simulink model "ADCSSimulator"  (R2024a)
settings: Solver=ode4  StartTime=0.0  StopTime=600  FixedStep=0.01  MaxStep=0.1  RelTol=1e-3  AbsTol=1e-3
values from neighbouring files (symbols this model uses):
  ActuatorAllocationMatrix = ActuatorPhysicalMatrix' * inv(ActuatorPhysicalMatrix * ActuatorPhysicalMatrix')    [set_Init.m]
  ActuatorPhysicalMatrix = [1, 0, 0, 0 ... (first row only)    [set_Init.m]
  albedo_irradiance = 300    [set_Init.m]
  b = 0    [set_Init.m]
  Cd = 2.2    [set_Init.m]
  h_bias = [0; 0; 0]    [set_Init.m]
  J = 4.0e-3 / 628    (= 6.36942675159e-06)    [set_Init.m]
  k_Bdot = ((4 * pi * 0.5236 * 0.0055) / (5677.2 * (4.5e-5)^2))    (= 3147.8423197)    [set_Init.m]
  K_E = K_T    (= 0.0022)    [set_Init.m]
  K_T = 0.0022    [set_Init.m]
  P0 = blkdiag(P0_att, P0_bias)    [set_Init.m]
  P0_att = eye(3) * initial_variance_rad2    [set_Init.m]
  PowerVoltageBus_01 = 3.3    [set_Init.m]
  PowerVoltageBus_02 = 3.3    [set_Init.m]
  PowerVoltageBus_03 = 3.3    [set_Init.m]
  PowerVoltageBus_04 = 3.3    [set_Init.m]
  PowerVoltageBus_05 = 3.3    [set_Init.m]
  PowerVoltageBus_06 = 3.3    [set_Init.m]
  PowerVoltageBus_07 = 3.3    [set_Init.m]
  PowerVoltageBus_08 = 3.3    [set_Init.m]
  PowerVoltageBus_09 = 3.3    [set_Init.m]
  PowerVoltageBus_10 = 3.3    [set_Init.m]
  PowerVoltageBus_11 = 3.3    [set_Init.m]
  PowerVoltageBus_12 = 0.0    (= 0)    [set_Init.m]
  PowerVoltageBus_13 = 0.0    (= 0)    [set_Init.m]
  PowerVoltageBus_14 = 0.0    (= 0)    [set_Init.m]
  PowerVoltageBus_15 = 0.0    (= 0)    [set_Init.m]
  R = 2.0    (= 2)    [set_Init.m]
  ressidual_m = [3e-4; -2e-4; 1e-4]    [set_Init.m]
  solar_irradiance = 1361    [set_Init.m]
  surface_areas = [A_xy, A_yz, A_xz, A_xy, A_yz, A_xz]    [set_Init.m]
  surface_normals_body = [eye(3) -eye(3)]    [set_Init.m]
  surface_positions_body = [       hx,   0,   0 ... (first row only)    [set_Init.m]
  surface_reflectivities = [0.9 0.8 0.9 0.9 0.9 0.9]    [set_Init.m]
  Switch_01 = 1    [set_Init.m]
  Switch_02 = 1    [set_Init.m]
  Switch_03 = 1    [set_Init.m]
  Switch_04 = 1    [set_Init.m]
  Switch_05 = 1    [set_Init.m]
  Switch_06 = 1    [set_Init.m]
  Switch_07 = 1    [set_Init.m]
  Switch_08 = 1    [set_Init.m]
  Switch_09 = 1    [set_Init.m]
  Switch_10 = 1    [set_Init.m]
  Switch_11 = 1    [set_Init.m]
  Switch_12 = 0    [set_Init.m]
  Switch_13 = 0    [set_Init.m]
  Switch_14 = 0    [set_Init.m]
  Switch_15 = 0    [set_Init.m]
  visSampleTime = 0.1    [set_Init.m]
undefined symbols (not defined in the file or in its folder): attitude, Controller, epoch, IAU, juliandate, Kd, km, Kp, m, rad, s, satellite, SGP4_parameters, simulator, UKF_parameters, WMM2020
libraries: sharedtransform x27, aerolibutil x22, aerolibconvert2 x18, simulink_extras x16, matrix_library x6, aerolibtransform2 x4, vrlib x2, aerolibgravity2 x2, aerolibobsolete x1, aerolibattitudesys x1, simulink x1
(part 4 of 8)

== system ADCSSimulator/ADCS/ADCS Software/Onboard Reference Frames Transformations Manager1/Ensure Quaternion Continuity3 ==
  q_in : Inport
  Ensure Quaternion Continuity : MATLAB Function  TreatAsAtomicUnit=on
  Unit Delay : UnitDelay  InitialCondition=[1;0;0;0]  SampleTime=-1  HasFrameUpgradeWarning=on
  q_out : Outport
  wires:
  Ensure Quaternion Continuity/1(q_out) -> q_out/1, Unit Delay/1
  Unit Delay/1 -> Ensure Quaternion Continuity/2(q_prev)
  q_in/1 -> Ensure Quaternion Continuity/1(q_new)

== system ADCSSimulator/ADCS/ADCS Software/Onboard Reference Frames Transformations Manager1/Ensure Quaternion Continuity4 ==
  q_in : Inport
  Ensure Quaternion Continuity : MATLAB Function  TreatAsAtomicUnit=on
  Unit Delay : UnitDelay  InitialCondition=[1;0;0;0]  SampleTime=-1  HasFrameUpgradeWarning=on
  q_out : Outport
  wires:
  Ensure Quaternion Continuity/1(q_out) -> q_out/1, Unit Delay/1
  Unit Delay/1 -> Ensure Quaternion Continuity/2(q_prev)
  q_in/1 -> Ensure Quaternion Continuity/1(q_new)

== system ADCSSimulator/ADCS/ADCS Software/Onboard Reference Frames Transformations Manager1/Ensure Quaternion Continuity5 ==
  q_in : Inport
  Ensure Quaternion Continuity : MATLAB Function  TreatAsAtomicUnit=on
  Unit Delay : UnitDelay  InitialCondition=[1;0;0;0]  SampleTime=-1  HasFrameUpgradeWarning=on
  q_out : Outport
  wires:
  Ensure Quaternion Continuity/1(q_out) -> q_out/1, Unit Delay/1
  Unit Delay/1 -> Ensure Quaternion Continuity/2(q_prev)
  q_in/1 -> Ensure Quaternion Continuity/1(q_new)

== system ADCSSimulator/ADCS/ADCS Software/Onboard Reference Frames Transformations Manager1/ICRF to ITRF DCM Calculator ==
  note: Goal: Transformation Between ICRF (ECI) and ITRF (ECEF)
  note: **********************************************************************
      | * *
      | * I E R S B U L L E T I N - A *
      | * *
      | * Rapid Service/Prediction of Earth Orientation *
      | **********************************************************************
      | 30 September 2021 Vol. XXXIV No. 039
      | ______________________________________________________________________
      | GENERAL INFORMATION:
      | To receive this information electronically, contact:
      | ser7@maia.usno.navy.mil or use
      | <http://maia.usno.navy.mil/docrequest.html>
      | MJD = Julian Date - 2 400 000.5 days
      | UT2-UT1 = 0.022 sin(2*pi*T) - 0.012 cos(2*pi*T)
      | - 0.006 sin(4*pi*T) + 0.007 cos(4*pi*T)
      | where pi = 3.14159265... and T is the date in Besselian years.
      | TT = TAI + 32.184 seconds
      | DUT1= (UT1-UTC) transmitted with time signals
      | = -0.1 seconds beginning 17 July 2021 at 0000 UTC
      | Beginning 1 January 2017:
      | TAI-UTC = 37.000 000 seconds
  Calendar : Inport
  Bus Selector : BusSelector  OutputSignals=Modified Julian Date (day),Since Epoch (sec)
  Constant2 : Constant  Value=37
  Direction Cosine Matrix ICRF to ITRF : aerolibtransform2/Direction Cosine Matrix ECI to ECEF  red=IAU-2000/2006  year=epoch.Year  month=October  day=12  hour=epoch.Hour  min=epoch.Minute  sec=epoch.Second  deltaT=Sec  errorflag=Error  extraparamflag=on
      settings: AttributesFormatString=%<red>
  Earth Orientation Parameters : EOParameters
  ICRF to ITRF DCM : Outport
  wires:
  Earth Orientation Parameters/2 -> Direction Cosine Matrix ICRF to ITRF/3  "Polar Displacement of Earth"
  Constant2/1 -> Direction Cosine Matrix ICRF to ITRF/2
  Calendar/1 -> Bus Selector/1
  Earth Orientation Parameters/3 -> Direction Cosine Matrix ICRF to ITRF/4  "Celestial Intermediate Pole (CIP)  adjustment (radians)"
  Direction Cosine Matrix ICRF to ITRF/1 -> ICRF to ITRF DCM/1
  Bus Selector/1 -> Earth Orientation Parameters/1  "<Modified Julian Date (day)>"
  Earth Orientation Parameters/1 -> Direction Cosine Matrix ICRF to ITRF/1
  Bus Selector/2 -> Direction Cosine Matrix ICRF to ITRF/5  "<Since Epoch (sec)>"

== system ADCSSimulator/ADCS/ADCS Software/Onboard Reference Frames Transformations Manager1/Orbit to Body Transfer Matrix Calculator1 ==
  ICRF2BodyDCM : Inport
  Keplerian Elements : Inport  Port=2
  Bus Selector : BusSelector  OutputSignals=Argument of Perigee [omega] (rad),True Anomaly [nu] (rad),Inclination [i] (rad),Right Ascension [Omega] (rad)
  Interpreted MATLAB Function : MATLABFcn  MATLABFcn=[cos(u),sin(u),0; -sin(u),cos(u),0; 0,0,1]  OutputDimensions=[3,3]  Output1D=off
  Interpreted MATLAB Function1 : MATLABFcn  MATLABFcn=[1,0,0;0,cos(u),sin(u);0,-sin(u),cos(u)]  OutputDimensions=[3,3]  Output1D=off
  Interpreted MATLAB Function2 : MATLABFcn  MATLABFcn=[cos(u),sin(u),0;-sin(u),cos(u),0;0,0,1]  OutputDimensions=[3,3]  Output1D=off
  Matrix Multiply{,1..3} (4 alike) : Product  Multiplication=Matrix(*)
  RotMat : Constant  Value=[0,1,0;0,0,-1;-1,0,0]
  Sum : Sum  Inputs=|++
  Transpose : Math  Operator=transpose
  Orbit2BodyTM : Outport
  wires:
  Bus Selector/3 -> Interpreted MATLAB Function1/1  "<Inclination [i] (rad)>"
  Keplerian Elements/1 -> Bus Selector/1
  Interpreted MATLAB Function2/1 -> Matrix Multiply1/2
  Interpreted MATLAB Function/1 -> Matrix Multiply/1
  Sum/1 -> Interpreted MATLAB Function/1
  RotMat/1 -> Matrix Multiply2/1
  Matrix Multiply2/1 -> Transpose/1  "ICRF to Orbit DCM"
  ICRF2BodyDCM/1 -> Matrix Multiply3/1  "ICRF to Body DCM"
  Bus Selector/1 -> Sum/1  "<Argument of Perigee [omega] (rad)>"
  Bus Selector/2 -> Sum/2  "<True Anomaly [nu] (rad)>"
  Matrix Multiply/1 -> Matrix Multiply1/1
  Matrix Multiply3/1 -> Orbit2BodyTM/1  "Orbit to Body DCM"
  Interpreted MATLAB Function1/1 -> Matrix Multiply/2
  Bus Selector/4 -> Interpreted MATLAB Function2/1  "<Right Ascension [Omega] (rad)>"
  Matrix Multiply1/1 -> Matrix Multiply2/2  "ICRF to Orbit DCM"
  Transpose/1 -> Matrix Multiply3/2  "Orbit to ICRF DCM"

== system ADCSSimulator/ADCS/ADCS Software/Orbit Detemination/Latching Logic ==
  Satellite Postion [ICRF] (km) : Inport
  Satellite Velocity [ICRF] (km/s) : Inport  Port=2
  Clock : Clock
  MATLAB Function4 : MATLAB Function  TreatAsAtomicUnit=on
  Switch : Switch  Criteria=u2 > Threshold  SaturateOnIntegerOverflow=off  InputSameDT=off
  Unit Delay : UnitDelay  InitialCondition=zeros(6, 1)  SampleTime=-1  HasFrameUpgradeWarning=on
  x_initial : Outport
  wires:
  Satellite Velocity [ICRF] (km/s)/1 -> MATLAB Function4/2(v_eci_km_s)
  Satellite Postion [ICRF] (km)/1 -> MATLAB Function4/1(r_eci_km)
  Clock/1 -> Switch/2
  MATLAB Function4/1(x_initial) -> Switch/3
  Switch/1 -> Unit Delay/1
  Unit Delay/1 -> Switch/1, x_initial/1

== system ADCSSimulator/ADCS/ADCS Software/Orbit Detemination/Onboard Orbit Propagator  ==
  Measured Satellite Ephemeris : Inport
  Bus Creator4 : BusCreator  Inputs=4
  Bus Selector4 : BusSelector  OutputSignals=Measured Position [ITRF] (m),Measured Velocity [ITRF] (m/s)
  Orbit Propagator Numerical (Kepler-Unperturbed) : OrbitPropagator  propagator=Numerical (high precision)  startDate=juliandate(epoch.Year, epoch.Month, epoch.Day, epoch.Hour, epoch.Minute, epoch.Second)  dateOut=off  orbitType=Circular inclined  semiMajorAxis=Semi_major_axis  inclination=Inclination  raan=RAAN  argLat=Argument_of_latitude  inertialPosition=[3649700.0 3308200.0 -4676600.0]  inertialVelocity=[-2750.8 6666.4 2573.4]  fixedPosition=[-4142689.0 -2676864.7 -4669861.6]  fixedVelocity=[1452.7 -6720.7 2568.1]  customR=3396200  customMu=4.305e13  customJ2=1.0826269e-03  customOmega=4.06125949e-3
  Onboard Satellite Ephemeris [ICRF] : Outport
  wires:
  Orbit Propagator Numerical (Kepler-Unperturbed)/2 -> Bus Creator4/2  "Satellite Velocity [ICRF] (m/s)"
  Orbit Propagator Numerical (Kepler-Unperturbed)/1 -> Bus Creator4/1  "Satellite Position [ICRF] (m)"
  Bus Creator4/1 -> Onboard Satellite Ephemeris [ICRF]/1  "Onboard Satellite Ephemeris [ICRF]"
  Measured Satellite Ephemeris/1 -> Bus Selector4/1
  Bus Selector4/1 -> Bus Creator4/3  "<Measured Position [ITRF] (m)>"
  Bus Selector4/2 -> Bus Creator4/4  "<Measured Velocity [ITRF] (m/s)>"

== system ADCSSimulator/ADCS/ADCS Software/Orbit Detemination/Step Time ==
  Add : Sum  Inputs=|+-
  Clock : Clock
  Unit Delay : UnitDelay  SampleTime=-1  HasFrameUpgradeWarning=on
  dt : Outport
  wires:
  Clock/1 -> Unit Delay/1, Add/1
  Add/1 -> dt/1
  Unit Delay/1 -> Add/2

== system ADCSSimulator/ADCS/ADCS Software/Orbit Detemination/Step Time1 ==
  Add : Sum  Inputs=|+-
  Clock : Clock
  Unit Delay : UnitDelay  SampleTime=-1  HasFrameUpgradeWarning=on
  dt : Outport
  wires:
  Unit Delay/1 -> Add/2
  Add/1 -> dt/1
  Clock/1 -> Add/1, Unit Delay/1

== system ADCSSimulator/ADCS/Environment Model/Attitude Dynamics & Kynematics/sqrt ==
  u : Inport
  Dot Product : DotProduct  OutDataTypeStr=Inherit: Inherit via internal rule
  Sqrt1 : Sqrt
  sqrt(u) : Outport
  wires:
  Dot Product/1 -> Sqrt1/1
  u/1 -> Dot Product/2, Dot Product/1
  Sqrt1/1 -> sqrt(u)/1

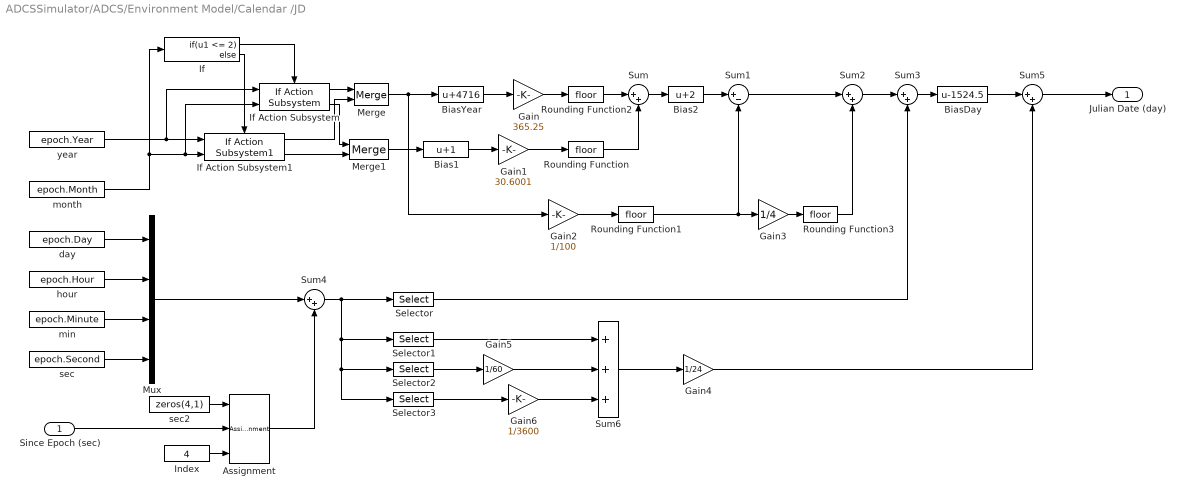
== system ADCSSimulator/ADCS/Environment Model/Calendar /JD ==
  Since Epoch (sec) : Inport  OutMin=0  PortDimensions=1
  Assignment : Assignment  IndexOptions=Index vector (port)  Indices=1  OutputSizes=1
  Bias1 : Bias  Bias=1  SaturateOnIntegerOverflow=off
  Bias2 : Bias  Bias=2  SaturateOnIntegerOverflow=off
  BiasDay : Bias  Bias=-1524.5  SaturateOnIntegerOverflow=off
  BiasYear : Bias  Bias=4716  SaturateOnIntegerOverflow=off
  Gain : Gain  Gain=365.25
  Gain1 : Gain  Gain=30.6001
  Gain2 : Gain  Gain=1/100
  Gain3 : Gain  Gain=1/4
  Gain4 : Gain  Gain=1/24
  Gain5 : Gain  Gain=1/60
  Gain6 : Gain  Gain=1/3600
  If : If  IfExpression=u1 <= 2
  If Action Subsystem : aerolibconvert2/Julian Date Conversion/If Action Subsystem  SystemSampleTime=-1  VariantActivationTime=update diagram  AllowFlexibleInterface=on  Latency=0  AutoFrameSizeCalculation=off
  If Action Subsystem1 : aerolibconvert2/Julian Date Conversion/If Action Subsystem1  SystemSampleTime=-1  VariantActivationTime=update diagram  AllowFlexibleInterface=on  Latency=0  AutoFrameSizeCalculation=off
  Index : Constant  Value=4
  Merge : Merge
  Merge1 : Merge
  Mux : Mux
  Rounding Function{,1..3} (4 alike) : Rounding
  Selector : Selector  InputPortWidth=4  IndexOptions=Index vector (dialog)  Indices=[1]  OutputSizes=1
  Selector1 : Selector  InputPortWidth=4  IndexOptions=Index vector (dialog)  Indices=[2]  OutputSizes=1
  Selector2 : Selector  InputPortWidth=4  IndexOptions=Index vector (dialog)  Indices=[3]  OutputSizes=1
  Selector3 : Selector  InputPortWidth=4  IndexOptions=Index vector (dialog)  Indices=[4]  OutputSizes=1
  Sum{,2..5} (5 alike) : Sum  Inputs=|++
  Sum1 : Sum  Inputs=|+-
  Sum6 : Sum  Inputs=+++
  day : Constant  Value=epoch.Day
  hour : Constant  Value=epoch.Hour
  min : Constant  Value=epoch.Minute
  month : Constant  Value=epoch.Month
  sec : Constant  Value=epoch.Second
  sec2 : Constant  Value=zeros(4,1)
  year : Constant  Value=epoch.Year
  Julian Date (day) : Outport  VectorParamsAs1DForOutWhenUnconnected=off
  wires:
  Merge1/1 -> Bias1/1
  Mux/1 -> Sum4/1
  month/1 -> If/1, If Action Subsystem1/2, If Action Subsystem/2
  Rounding Function/1 -> Sum/2
  day/1 -> Mux/1
  If Action Subsystem1/2 -> Merge1/2
  Sum/1 -> Bias2/1
  Sum6/1 -> Gain4/1
  BiasDay/1 -> Sum5/1
  hour/1 -> Mux/2
  Selector/1 -> Sum3/2
  sec/1 -> Mux/4
  Since Epoch (sec)/1 -> Assignment/2
  If/2 -> If Action Subsystem1/Action
  Rounding Function1/1 -> Sum1/2, Gain3/1
  Gain5/1 -> Sum6/2
  Assignment/1 -> Sum4/2
  Bias2/1 -> Sum1/1
  Gain/1 -> Rounding Function2/1
  Gain2/1 -> Rounding Function1/1
  Sum4/1 -> Selector/1, Selector3/1, Selector2/1, Selector1/1
  If Action Subsystem/1 -> Merge/1
  year/1 -> If Action Subsystem1/1, If Action Subsystem/1
  Gain6/1 -> Sum6/3
  Sum3/1 -> BiasDay/1
  If Action Subsystem/2 -> Merge1/1
  Bias1/1 -> Gain1/1
  Rounding Function3/1 -> Sum2/2
  Gain1/1 -> Rounding Function/1
  sec2/1 -> Assignment/1
  Sum1/1 -> Sum2/1
  Sum5/1 -> Julian Date (day)/1
  Selector1/1 -> Sum6/1
  Sum2/1 -> Sum3/1
  Gain4/1 -> Sum5/2
  BiasYear/1 -> Gain/1
  Merge/1 -> BiasYear/1, Gain2/1
  Gain3/1 -> Rounding Function3/1
  Selector2/1 -> Gain5/1
  Rounding Function2/1 -> Sum/1
  Selector3/1 -> Gain6/1
  If/1 -> If Action Subsystem/Action
  min/1 -> Mux/3
  If Action Subsystem1/1 -> Merge/2
  Index/1 -> Assignment/3

== system ADCSSimulator/ADCS/Environment Model/Calendar /MJD ==
  Since Epoch (sec) : Inport  OutMin=0  PortDimensions=1
  Assignment : Assignment  IndexOptions=Index vector (port)  Indices=1  OutputSizes=1
  Bias1 : Bias  Bias=1  SaturateOnIntegerOverflow=off
  Bias2 : Bias  Bias=2  SaturateOnIntegerOverflow=off
  BiasDay : Bias  Bias=-679006  SaturateOnIntegerOverflow=off
  BiasYear : Bias  SaturateOnIntegerOverflow=off
  Gain : Gain  Gain=365.25
  Gain1 : Gain  Gain=30.6001
  Gain2 : Gain  Gain=1/100
  Gain3 : Gain  Gain=1/4
  Gain4 : Gain  Gain=1/24
  Gain5 : Gain  Gain=1/60
  Gain6 : Gain  Gain=1/3600
  If : If  IfExpression=u1 <= 2
  If Action Subsystem : aerolibconvert2/Julian Date Conversion/If Action Subsystem  SystemSampleTime=-1  VariantActivationTime=update diagram  AllowFlexibleInterface=on  Latency=0  AutoFrameSizeCalculation=off
  If Action Subsystem1 : aerolibconvert2/Julian Date Conversion/If Action Subsystem1  SystemSampleTime=-1  VariantActivationTime=update diagram  AllowFlexibleInterface=on  Latency=0  AutoFrameSizeCalculation=off
  Index : Constant  Value=4
  Merge : Merge
  Merge1 : Merge
  Mux : Mux
  Rounding Function{,1..3} (4 alike) : Rounding
  Selector : Selector  InputPortWidth=4  IndexOptions=Index vector (dialog)  Indices=[1]  OutputSizes=1
  Selector1 : Selector  InputPortWidth=4  IndexOptions=Index vector (dialog)  Indices=[2]  OutputSizes=1
  Selector2 : Selector  InputPortWidth=4  IndexOptions=Index vector (dialog)  Indices=[3]  OutputSizes=1
  Selector3 : Selector  InputPortWidth=4  IndexOptions=Index vector (dialog)  Indices=[4]  OutputSizes=1
  Sum{,2..5} (5 alike) : Sum  Inputs=|++
  Sum1 : Sum  Inputs=|+-
  Sum6 : Sum  Inputs=+++
  day : Constant  Value=epoch.Day
  hour : Constant  Value=epoch.Hour
  min : Constant  Value=epoch.Minute
  month : Constant  Value=epoch.Month
  sec : Constant  Value=epoch.Second
  sec2 : Constant  Value=zeros(4,1)
  year : Constant  Value=epoch.Year
  Modified Julian Date (day) : Outport  VectorParamsAs1DForOutWhenUnconnected=off
  wires:
  Rounding Function/1 -> Sum/2
  If/2 -> If Action Subsystem1/Action
  Gain4/1 -> Sum5/2
  BiasYear/1 -> Gain/1
  Bias2/1 -> Sum1/1
  Selector1/1 -> Sum6/1
  Sum/1 -> Bias2/1
  Sum2/1 -> Sum3/1
  BiasDay/1 -> Sum5/1
  Selector/1 -> Sum3/2
  Sum1/1 -> Sum2/1
  year/1 -> If Action Subsystem1/1, If Action Subsystem/1
  Sum5/1 -> Modified Julian Date (day)/1
  Sum6/1 -> Gain4/1
  hour/1 -> Mux/2
  Gain/1 -> Rounding Function2/1
  Merge1/1 -> Bias1/1
  Since Epoch (sec)/1 -> Assignment/2
  Gain6/1 -> Sum6/3
  Gain2/1 -> Rounding Function1/1
  Mux/1 -> Sum4/1
  Rounding Function1/1 -> Sum1/2, Gain3/1
  Rounding Function3/1 -> Sum2/2
  Sum3/1 -> BiasDay/1
  Selector3/1 -> Gain6/1
  Rounding Function2/1 -> Sum/1
  Gain1/1 -> Rounding Function/1
  sec2/1 -> Assignment/1
  day/1 -> Mux/1
  Bias1/1 -> Gain1/1
  min/1 -> Mux/3
  Gain3/1 -> Rounding Function3/1
  If/1 -> If Action Subsystem/Action
  Gain5/1 -> Sum6/2
  If Action Subsystem1/1 -> Merge/2
  Sum4/1 -> Selector/1, Selector3/1, Selector2/1, Selector1/1
  Merge/1 -> BiasYear/1, Gain2/1
  If Action Subsystem/1 -> Merge/1
  Selector2/1 -> Gain5/1
  If Action Subsystem/2 -> Merge1/1
  month/1 -> If/1, If Action Subsystem1/2, If Action Subsystem/2
  sec/1 -> Mux/4
  If Action Subsystem1/2 -> Merge1/2
  Assignment/1 -> Sum4/2
  Index/1 -> Assignment/3

== system ADCSSimulator/ADCS/Environment Model/Disturbance Calculator/Aerodynamic Torque ==
  Satellite Positon [Body](m) : Inport
  Satellite Velocity [Body](m/s) : Inport  Port=2
  Drag coefficient : Constant  Value=Cd
  MATLAB Function1 : MATLAB Function  TreatAsAtomicUnit=on
  Matrix of Center-of-Pressure Positions in Body Frame [m] : Constant  Value=surface_positions_body
  Matrix of Surface Normals in Body Frame : Constant  Value=surface_normals_body
  Vector of Surface Areas [m²] : Constant  Value=surface_areas
  Aerodynamics Drag Torque [Body](N.m) : Outport
  wires:
  Satellite Positon [Body](m)/1 -> MATLAB Function1/1(R_body)
  Satellite Velocity [Body](m/s)/1 -> MATLAB Function1/2(V_body)
  Matrix of Surface Normals in Body Frame/1 -> MATLAB Function1/3(surface_normals)
  Vector of Surface Areas [m²]/1 -> MATLAB Function1/4(surface_areas)
  Matrix of Center-of-Pressure Positions in Body Frame [m]/1 -> MATLAB Function1/5(surface_positions)
  Drag coefficient/1 -> MATLAB Function1/6(Cd)
  MATLAB Function1/1(aerodynamic_drag_torque) -> Aerodynamics Drag Torque [Body](N.m)/1

== system ADCSSimulator/ADCS/Environment Model/Disturbance Calculator/Gravity Gradient ==
  Satellite Positon [Body](m) : Inport
  Constant1 : Constant  Value=satellite.MOI
  MATLAB Function : MATLAB Function  TreatAsAtomicUnit=on
  Gravity Gradient [Body](N.m) : Outport
  wires:
  Constant1/1 -> MATLAB Function/2(J)
  MATLAB Function/1(gravity_gradient_torque) -> Gravity Gradient [Body](N.m)/1
  Satellite Positon [Body](m)/1 -> MATLAB Function/1(Rearth_body)

== system ADCSSimulator/ADCS/Environment Model/Disturbance Calculator/Magnetic Field Disturbance ==
  Magnetic Field [Body](T) : Inport
  Cross Product : matrix_library/Cross Product
  Residual Magnetic Dipole (A.m^2) : Constant  Value=ressidual_m
  Magnetic Field Disturbance [Body](N.m) : Outport
  wires:
  Magnetic Field [Body](T)/1 -> Cross Product/2
  Cross Product/1 -> Magnetic Field Disturbance [Body](N.m)/1
  Residual Magnetic Dipole (A.m^2)/1 -> Cross Product/1

== system ADCSSimulator/ADCS/Environment Model/Disturbance Calculator/Solar Radiation Pressure (SRP) ==
  Sun Position [Body](m) : Inport
  Earth Position [Body](m) : Inport  Port=2
  Eclipse : Inport  Port=3
  Bus Creator : BusCreator  Inputs=2
  Bus Creator1 : BusCreator  Inputs=2
  Constant : Constant  Value=[0;0;0]
  Constant1 : Constant  Value=[0;0;0]
  Eclipse1 : InportShadow  Port=3
  MATLAB Function : MATLAB Function  TreatAsAtomicUnit=on
  MATLAB Function1 : MATLAB Function  TreatAsAtomicUnit=on
  MATLAB Function2 : MATLAB Function  TreatAsAtomicUnit=on
  Matrix of Center-of-Pressure Positions in Body Frame [m] : Constant  Value=surface_positions_body
  Matrix of Surface Normals in Body Frame : Constant  Value=surface_normals_body
  Solar Constant at Current Distance (e.g. 1361 W/m²) : Constant  Value=solar_irradiance
  Sum : Sum
  Switch : Switch  Criteria=u2 > Threshold  SaturateOnIntegerOverflow=off  InputSameDT=off
  Switch1 : Switch  Criteria=u2 > Threshold  SaturateOnIntegerOverflow=off  InputSameDT=off
  Vector of Surface Areas [m²] : Constant  Value=surface_areas
  Vector of Surface Reflectivity Coefficients [0 to 1] : Constant  Value=surface_reflectivities
  irradiance due to albedo : Constant  Value=albedo_irradiance
  Rediation Pressure Torques : Outport
  wires:
  Vector of Surface Reflectivity Coefficients [0 to 1]/1 -> MATLAB Function1/4(surface_reflectivities), MATLAB Function/4(surface_reflectivities)
  Sun Position [Body](m)/1 -> MATLAB Function/1(sun_vector_body)
  Matrix of Center-of-Pressure Positions in Body Frame [m]/1 -> MATLAB Function1/5(surface_positions_body), MATLAB Function/5(surface_positions_body)
  Vector of Surface Areas [m²]/1 -> MATLAB Function1/3(surface_areas), MATLAB Function/3(surface_areas)
  Matrix of Surface Normals in Body Frame/1 -> MATLAB Function1/2(surface_normals_body), MATLAB Function/2(surface_normals_body)
  irradiance due to albedo/1 -> MATLAB Function1/6(albedo_irradiance)
  Sum/1 -> Bus Creator/2  "Total Rediation Pressure Torque [Body](Nm)"
  Earth Position [Body](m)/1 -> MATLAB Function1/1(earth_vector_body), MATLAB Function2/1(earth_vector_body)
  Solar Constant at Current Distance (e.g. 1361 W/m²)/1 -> MATLAB Function/6(solar_irradiance)
  MATLAB Function/1(SRP_Torque) -> Switch/3
  MATLAB Function2/1(albedo_direction_body) -> MATLAB Function1/7(albedo_direction_body)
  Bus Creator/1 -> Rediation Pressure Torques/1
  Bus Creator1/1 -> Bus Creator/1  "Individuals Solar Rediation Torques [Body](N.m)"
  Constant/1 -> Switch/1
  Eclipse/1 -> Switch/2
  Switch/1 -> Sum/1, Bus Creator1/1  "Solar Rediation Pressure Torque [Body](Nm)"
  Eclipse1/1 -> Switch1/2
  Constant1/1 -> Switch1/1
  MATLAB Function1/1(albedo_RP_torque) -> Switch1/3
  Switch1/1 -> Sum/2, Bus Creator1/2  "Albedo Rediation Pressure Torque [Body](Nm)"

== system ADCSSimulator/ADCS/Environment Model/Reference Frames Transformations Manager/ICRF to Body Transfer Matrix Calculator ==
  Orbit2BodyDCM : Inport
  Keplerian Elements : Inport  Port=2
  Bus Selector : BusSelector  OutputSignals=Argument of Perigee [omega] (rad),True Anomaly [nu] (rad),Inclination [i] (rad),Right Ascension [Omega] (rad)
  Interpreted MATLAB Function : MATLABFcn  MATLABFcn=[cos(u),sin(u),0; -sin(u),cos(u),0; 0,0,1]  OutputDimensions=[3,3]  Output1D=off
  Interpreted MATLAB Function1 : MATLABFcn  MATLABFcn=[1,0,0;0,cos(u),sin(u);0,-sin(u),cos(u)]  OutputDimensions=[3,3]  Output1D=off
  Interpreted MATLAB Function2 : MATLABFcn  MATLABFcn=[cos(u),sin(u),0;-sin(u),cos(u),0;0,0,1]  OutputDimensions=[3,3]  Output1D=off
  Matrix Multiply{,1..3} (4 alike) : Product  Multiplication=Matrix(*)
  RotMat : Constant  Value=[0,1,0;0,0,-1;-1,0,0]
  Sum : Sum  Inputs=|++
  ICRF2BodyTM : Outport
  wires:
  Bus Selector/3 -> Interpreted MATLAB Function1/1  "<Inclination [i] (rad)>"
  Keplerian Elements/1 -> Bus Selector/1
  Interpreted MATLAB Function2/1 -> Matrix Multiply1/2
  Interpreted MATLAB Function/1 -> Matrix Multiply/1
  Sum/1 -> Interpreted MATLAB Function/1
  RotMat/1 -> Matrix Multiply2/1
  Matrix Multiply2/1 -> Matrix Multiply3/2  "ICRF to Orbit DCM"
  Orbit2BodyDCM/1 -> Matrix Multiply3/1  "Orbit to Body DCM"
  Bus Selector/1 -> Sum/1  "<Argument of Perigee [omega] (rad)>"
  Bus Selector/2 -> Sum/2  "<True Anomaly [nu] (rad)>"
  Matrix Multiply/1 -> Matrix Multiply1/1
  Matrix Multiply3/1 -> ICRF2BodyTM/1  "ICRF to Body DCM"
  Interpreted MATLAB Function1/1 -> Matrix Multiply/2
  Bus Selector/4 -> Interpreted MATLAB Function2/1  "<Right Ascension [Omega] (rad)>"
  Matrix Multiply1/1 -> Matrix Multiply2/2  "ICRF to Orbit DCM"

== system ADCSSimulator/ADCS/Environment Model/Reference Frames Transformations Manager/ICRF to ITRF DCM Calculator ==
  note: Goal: Transformation Between ICRF (ECI) and ITRF (ECEF)
  note: **********************************************************************
      | * *
      | * I E R S B U L L E T I N - A *
      | * *
      | * Rapid Service/Prediction of Earth Orientation *
      | **********************************************************************
      | 30 September 2021 Vol. XXXIV No. 039
      | ______________________________________________________________________
      | GENERAL INFORMATION:
      | To receive this information electronically, contact:
      | ser7@maia.usno.navy.mil or use
      | <http://maia.usno.navy.mil/docrequest.html>
      | MJD = Julian Date - 2 400 000.5 days
      | UT2-UT1 = 0.022 sin(2*pi*T) - 0.012 cos(2*pi*T)
      | - 0.006 sin(4*pi*T) + 0.007 cos(4*pi*T)
      | where pi = 3.14159265... and T is the date in Besselian years.
      | TT = TAI + 32.184 seconds
      | DUT1= (UT1-UTC) transmitted with time signals
      | = -0.1 seconds beginning 17 July 2021 at 0000 UTC
      | Beginning 1 January 2017:
      | TAI-UTC = 37.000 000 seconds
  Calendar : Inport
  Bus Selector : BusSelector  OutputSignals=Modified Julian Date (day),Since Epoch (sec)
  Constant2 : Constant  Value=37
  Direction Cosine Matrix ICRF to ITRF : aerolibtransform2/Direction Cosine Matrix ECI to ECEF  red=IAU-2000/2006  year=epoch.Year  month=October  day=12  hour=epoch.Hour  min=epoch.Minute  sec=epoch.Second  deltaT=Sec  errorflag=Error  extraparamflag=on
      settings: AttributesFormatString=%<red>
  Earth Orientation Parameters : EOParameters
  ICRF to ITRF DCM : Outport
  wires:
  Earth Orientation Parameters/2 -> Direction Cosine Matrix ICRF to ITRF/3  "Polar Displacement of Earth"
  Constant2/1 -> Direction Cosine Matrix ICRF to ITRF/2
  Calendar/1 -> Bus Selector/1
  Earth Orientation Parameters/3 -> Direction Cosine Matrix ICRF to ITRF/4  "Celestial Intermediate Pole (CIP)  adjustment (radians)"
  Direction Cosine Matrix ICRF to ITRF/1 -> ICRF to ITRF DCM/1
  Bus Selector/1 -> Earth Orientation Parameters/1  "<Modified Julian Date (day)>"
  Earth Orientation Parameters/1 -> Direction Cosine Matrix ICRF to ITRF/1
  Bus Selector/2 -> Direction Cosine Matrix ICRF to ITRF/5  "<Since Epoch (sec)>"

== system ADCSSimulator/ADCS/Environment Model/Reference Frames Transformations Manager/Quaternion Conditioner ==
  Q : Inport  PortDimensions=[4,1]
  Interpreted MATLAB Function : MATLABFcn  MATLABFcn=[u(1),0,0,0;0,u(2),0,0;0,0,u(3),0;0,0,0,u(4)]
  Interpreted MATLAB Function1 : MATLABFcn  MATLABFcn=[u(1),0,0,0;0,u(2),0,0;0,0,u(3),0;0,0,0,u(4)]
  Interpreted MATLAB Function2 : MATLABFcn  MATLABFcn=(u(1)+u(6)+u(11)+u(16))+1.9
  Product : Product
  Product1 : Product
  Sign : Signum
  Sign1 : Signum
  Unit Delay : UnitDelay  InitialCondition=[1;0;0;0]  SampleTime=-1  HasFrameUpgradeWarning=on
  Qc : Outport  PortDimensions=[4,1]
  wires:
  Product1/1 -> Qc/1, Unit Delay/1
  Interpreted MATLAB Function/1 -> Product/1
  Interpreted MATLAB Function2/1 -> Sign1/1
  Sign/1 -> Interpreted MATLAB Function2/1
  Product/1 -> Sign/1
  Sign1/1 -> Product1/2
  Q/1 -> Interpreted MATLAB Function/1, Product1/1
  Interpreted MATLAB Function1/1 -> Product/2
  Unit Delay/1 -> Interpreted MATLAB Function1/1

== system ADCSSimulator/ADCS/Environment Model/Reference Frames Transformations Manager/Quaternion Conditioner0 ==
  Q : Inport  PortDimensions=[4,1]
  Interpreted MATLAB Function : MATLABFcn  MATLABFcn=[u(1),0,0,0;0,u(2),0,0;0,0,u(3),0;0,0,0,u(4)]
  Interpreted MATLAB Function1 : MATLABFcn  MATLABFcn=[u(1),0,0,0;0,u(2),0,0;0,0,u(3),0;0,0,0,u(4)]
  Interpreted MATLAB Function2 : MATLABFcn  MATLABFcn=(u(1)+u(6)+u(11)+u(16))+1.9
  Product : Product
  Product1 : Product
  Sign : Signum
  Sign1 : Signum
  Unit Delay : UnitDelay  InitialCondition=[1;0;0;0]  SampleTime=-1  HasFrameUpgradeWarning=on
  Qc : Outport  PortDimensions=[4,1]
  wires:
  Unit Delay/1 -> Interpreted MATLAB Function1/1
  Interpreted MATLAB Function1/1 -> Product/2
  Q/1 -> Product1/1, Interpreted MATLAB Function/1
  Sign1/1 -> Product1/2
  Product/1 -> Sign/1
  Sign/1 -> Interpreted MATLAB Function2/1
  Interpreted MATLAB Function2/1 -> Sign1/1
  Interpreted MATLAB Function/1 -> Product/1
  Product1/1 -> Unit Delay/1, Qc/1

== system ADCSSimulator/ADCS/Environment Model/Reference Frames Transformations Manager/Quaternion Conditioner1 ==
  Q : Inport  PortDimensions=[4,1]
  Interpreted MATLAB Function : MATLABFcn  MATLABFcn=[u(1),0,0,0;0,u(2),0,0;0,0,u(3),0;0,0,0,u(4)]
  Interpreted MATLAB Function1 : MATLABFcn  MATLABFcn=[u(1),0,0,0;0,u(2),0,0;0,0,u(3),0;0,0,0,u(4)]
  Interpreted MATLAB Function2 : MATLABFcn  MATLABFcn=(u(1)+u(6)+u(11)+u(16))+1.9
  Product : Product
  Product1 : Product
  Sign : Signum
  Sign1 : Signum
  Unit Delay : UnitDelay  InitialCondition=[1;0;0;0]  SampleTime=-1  HasFrameUpgradeWarning=on
  Qc : Outport  PortDimensions=[4,1]
  wires:
  Product1/1 -> Qc/1, Unit Delay/1
  Interpreted MATLAB Function/1 -> Product/1
  Interpreted MATLAB Function2/1 -> Sign1/1
  Sign/1 -> Interpreted MATLAB Function2/1
  Product/1 -> Sign/1
  Sign1/1 -> Product1/2
  Q/1 -> Interpreted MATLAB Function/1, Product1/1
  Interpreted MATLAB Function1/1 -> Product/2
  Unit Delay/1 -> Interpreted MATLAB Function1/1

== system ADCSSimulator/ADCS/Environment Model/Reference Frames Transformations Manager/Quaternion Conditioner2 ==
  Q : Inport  PortDimensions=[4,1]
  Interpreted MATLAB Function : MATLABFcn  MATLABFcn=[u(1),0,0,0;0,u(2),0,0;0,0,u(3),0;0,0,0,u(4)]
  Interpreted MATLAB Function1 : MATLABFcn  MATLABFcn=[u(1),0,0,0;0,u(2),0,0;0,0,u(3),0;0,0,0,u(4)]
  Interpreted MATLAB Function2 : MATLABFcn  MATLABFcn=(u(1)+u(6)+u(11)+u(16))+1.9
  Product : Product
  Product1 : Product
  Sign : Signum
  Sign1 : Signum
  Unit Delay : UnitDelay  InitialCondition=[1;0;0;0]  SampleTime=-1  HasFrameUpgradeWarning=on
  Qc : Outport  PortDimensions=[4,1]
  wires:
  Unit Delay/1 -> Interpreted MATLAB Function1/1
  Interpreted MATLAB Function1/1 -> Product/2
  Q/1 -> Product1/1, Interpreted MATLAB Function/1
  Sign1/1 -> Product1/2
  Product/1 -> Sign/1
  Sign/1 -> Interpreted MATLAB Function2/1
  Interpreted MATLAB Function2/1 -> Sign1/1
  Interpreted MATLAB Function/1 -> Product/1
  Product1/1 -> Unit Delay/1, Qc/1

== system ADCSSimulator/ADCS/Environment Model/Reference Frames Transformations Manager/Quaternion Conditioner3 ==
  Q : Inport  PortDimensions=[4,1]
  Interpreted MATLAB Function : MATLABFcn  MATLABFcn=[u(1),0,0,0;0,u(2),0,0;0,0,u(3),0;0,0,0,u(4)]
  Interpreted MATLAB Function1 : MATLABFcn  MATLABFcn=[u(1),0,0,0;0,u(2),0,0;0,0,u(3),0;0,0,0,u(4)]
  Interpreted MATLAB Function2 : MATLABFcn  MATLABFcn=(u(1)+u(6)+u(11)+u(16))+1.9
  Product : Product
  Product1 : Product
  Sign : Signum
  Sign1 : Signum
  Unit Delay : UnitDelay  InitialCondition=[1;0;0;0]  SampleTime=-1  HasFrameUpgradeWarning=on
  Qc : Outport  PortDimensions=[4,1]
  wires:
  Product1/1 -> Qc/1, Unit Delay/1
  Interpreted MATLAB Function/1 -> Product/1
  Interpreted MATLAB Function2/1 -> Sign1/1
  Sign/1 -> Interpreted MATLAB Function2/1
  Product/1 -> Sign/1
  Sign1/1 -> Product1/2
  Q/1 -> Interpreted MATLAB Function/1, Product1/1
  Interpreted MATLAB Function1/1 -> Product/2
  Unit Delay/1 -> Interpreted MATLAB Function1/1

== system ADCSSimulator/ADCS/Environment Model/Reference Frames Transformations Manager/Quaternion Conditioner4 ==
  Q : Inport  PortDimensions=[4,1]
  Interpreted MATLAB Function : MATLABFcn  MATLABFcn=[u(1),0,0,0;0,u(2),0,0;0,0,u(3),0;0,0,0,u(4)]
  Interpreted MATLAB Function1 : MATLABFcn  MATLABFcn=[u(1),0,0,0;0,u(2),0,0;0,0,u(3),0;0,0,0,u(4)]
  Interpreted MATLAB Function2 : MATLABFcn  MATLABFcn=(u(1)+u(6)+u(11)+u(16))+1.9
  Product : Product
  Product1 : Product
  Sign : Signum
  Sign1 : Signum
  Unit Delay : UnitDelay  InitialCondition=[1;0;0;0]  SampleTime=-1  HasFrameUpgradeWarning=on
  Qc : Outport  PortDimensions=[4,1]
  wires:
  Unit Delay/1 -> Interpreted MATLAB Function1/1
  Interpreted MATLAB Function1/1 -> Product/2
  Q/1 -> Product1/1, Interpreted MATLAB Function/1
  Sign1/1 -> Product1/2
  Product/1 -> Sign/1
  Sign/1 -> Interpreted MATLAB Function2/1
  Interpreted MATLAB Function2/1 -> Sign1/1
  Interpreted MATLAB Function/1 -> Product/1
  Product1/1 -> Unit Delay/1, Qc/1

== system ADCSSimulator/ADCS/Environment Model/Reference Frames Transformations Manager/Virtual Reality World ==
  ITRF to Body Quaternions : Inport
  ICRF to Body Quaternions : Inport  Port=2
  Sun Position [ICRF] (m) : Inport  Port=3
  Satellite Position [ITRF] (m) : Inport  Port=4
  Antenna Position to VRML : Subsystem
  Compute Antenna Properties : Subsystem
  Compute Earth Rotation Rate : Subsystem
  Compute Umbra Translation : Subsystem
  Constant3 : Constant
  Constant4 : Constant  Value=[0 0 7.292115146706979e-5]'
  Constant5 : Constant  Value=[0 0 1]
  KeepSunInView : Gain  Gain=1/10
  Quaternion Inverse : aerolibutil/Quaternion Inverse
  Quaternion Inverse1 : aerolibutil/Quaternion Inverse
  Quaternion Rotation : aerolibutil/Quaternion Rotation
  Quaternion Rotation1 : aerolibutil/Quaternion Rotation
  Quaternion Rotation2 : aerolibutil/Quaternion Rotation
  Quaternion between r_a and r_b : aerolibattitudesys/Quaternion between vectors
  Quaternion to VRML : Subsystem
  Quaternion to VRML1 : Subsystem
  Radar on/off : Subsystem
  Rate Transition{1..7} (7 alike) : RateTransition
  Sat Position to VRML : Subsystem
  Satellite Model Scaling : Subsystem
  Sum : Sum  Inputs=++|
  Sun Position to VRML : Subsystem
  VR Sink : vrlib/VR Sink  InstantiateOnLoad=on  SampleTime=visSampleTime  ViewEnable=on  RemoteChange=off  RemoteView=off  FieldsWritten=Earth.rotation.4.1.1.double#Satellite.rotation.4.1.1.double#Satellite.scale.3.1.1.double#Satellite.translation.3.1.1.double#AntennaCone.rotation.4.1.1.double#AntennaCone.scale.3.1.1.double#AntennaCone.translation.3.1.1.double#AntennaMaterial.transparency.1.1.1.double#Sun.translation.3.1.1.double#Umbra.rotation.4.1.1.double#Umbra.translation.3.1.1.double  WorldFileName=cubesatAnim.wrl  WorldDescription=CubeSat Orbit Animation  AutoView=on  VideoDimensions=[]  AllowVariableSize=off
  m to VRML : Gain  Gain=1e-6
  wires:
  Rate Transition6/1 -> VR Sink/2, VR Sink/5
  Quaternion to VRML/1(axis_angle) -> Rate Transition6/1
  Rate Transition5/1 -> VR Sink/7
  Rate Transition3/1 -> VR Sink/4
  Rate Transition7/1 -> VR Sink/1
  Constant4/1 -> Compute Earth Rotation Rate/1(EarthRot)
  Rate Transition2/1 -> VR Sink/10
  Rate Transition1/1 -> VR Sink/9
  Rate Transition4/1 -> VR Sink/11
  Sun Position [ICRF] (m)/1 -> Quaternion Rotation1/2
  ICRF to Body Quaternions/1 -> Quaternion Rotation1/1
  Compute Antenna Properties/2(AntennaTrans) -> Quaternion Rotation/2
  Compute Antenna Properties/1(AntennaScale) -> m to VRML/1
  Satellite Model Scaling/1(Out1) -> Compute Antenna Properties/1(SatScale), VR Sink/3
  Compute Umbra Translation/1(O) -> Rate Transition4/1
  KeepSunInView/1 -> Rate Transition1/1, Compute Umbra Translation/1(I)
  Quaternion to VRML1/1(axis_angle) -> Rate Transition2/1
  Radar on/off/1(Radar) -> VR Sink/8
  Sat Position to VRML/1(xVRML) -> Rate Transition3/1
  Compute Earth Rotation Rate/1(VRMLRot) -> Rate Transition7/1
  Antenna Position to VRML/1(xVRML) -> Rate Transition5/1
  m to VRML/1 -> VR Sink/6
  Constant5/1 -> Quaternion between r_a and r_b/1
  Quaternion between r_a and r_b/1 -> Quaternion to VRML1/1(q)
  Sun Position to VRML/1(xVRML) -> KeepSunInView/1
  Quaternion Inverse1/1 -> Quaternion Rotation2/1
  Quaternion Rotation1/1 -> Quaternion Rotation2/2
  Quaternion Rotation2/1 -> Quaternion between r_a and r_b/2, Sun Position to VRML/1(x)
  Quaternion Rotation/1 -> Sum/2
  Sum/1 -> Antenna Position to VRML/1(x)
  Quaternion Inverse/1 -> Quaternion Rotation/1
  Satellite Position [ITRF] (m)/1 -> Sum/1, Sat Position to VRML/1(x)
  Constant3/1 -> Radar on/off/1(NavMode)
  ITRF to Body Quaternions/1 -> Quaternion Inverse1/1, Quaternion Inverse/1, Quaternion to VRML/1(q)

== system ADCSSimulator/ADCS/ADCS Hardware/Actuators/Reaction Wheels Model (RWs)/Reaction Wheel Assembly ==
  RWs Voltage Bus (V) : Inport
  RW Command Torque [Body](N.m) : Inport  Port=2
  1-axis Reaction Wheel (RW#1) : Subsystem
  1-axis Reaction Wheel (RW#2) : Subsystem
  1-axis Reaction Wheel (RW#3) : Subsystem
  1-axis Reaction Wheel (RW#4) : Subsystem
  Actuator Allocation Matrix (4*3) : Constant  Value=ActuatorAllocationMatrix
  Actuator Physical Matrix (3*4) : Constant  Value=ActuatorPhysicalMatrix
  Bus Creator : BusCreator  Inputs=4
  Bus Creator1 : BusCreator  Inputs=4
  Bus Creator2 : BusCreator  Inputs=4
  Bus Selector1 : BusSelector  OutputSignals=Power Bus: RW#1 (signal 5),Power Bus: RW#2 (signal 6),Power Bus: RW#3 (signal 7),Power Bus: RW#4 (signal 8)
  Demux : Demux
  Matrix Multiply : Product  Multiplication=Matrix(*)
  Matrix Multiply1 : Product  Multiplication=Matrix(*)
  RWs Torque Out (Nm) : Outport
  RWs Angular Velocity (rad/s) : Outport  Port=2
  RWs Power Status : Outport  Port=3
  wires:
  RWs Voltage Bus (V)/1 -> Bus Selector1/1
  RW Command Torque [Body](N.m)/1 -> Matrix Multiply1/2
  Bus Selector1/1 -> 1-axis Reaction Wheel (RW#1)/2(RW Bus Voltage (V))  "<Power Bus: RW#1 (signal 5)>"
  Bus Selector1/2 -> 1-axis Reaction Wheel (RW#2)/2(RW Bus Voltage (V))  "<Power Bus: RW#2 (signal 6)>"
  Bus Selector1/3 -> 1-axis Reaction Wheel (RW#3)/2(RW Bus Voltage (V))  "<Power Bus: RW#3 (signal 7)>"
  Demux/3 -> 1-axis Reaction Wheel (RW#3)/1(Command Torque [Body](N.m))
  Demux/2 -> 1-axis Reaction Wheel (RW#2)/1(Command Torque [Body](N.m))
  Demux/1 -> 1-axis Reaction Wheel (RW#1)/1(Command Torque [Body](N.m))
  1-axis Reaction Wheel (RW#1)/1(RW Torque Out) -> Bus Creator/1  "RW#1 Torque Out (N.m)"
  1-axis Reaction Wheel (RW#2)/1(RW Torque Out) -> Bus Creator/2  "RW#2 Torque Out (N.m)"
  1-axis Reaction Wheel (RW#3)/1(RW Torque Out) -> Bus Creator/3  "RW#3 Torque Out (N.m)"
  1-axis Reaction Wheel (RW#1)/2(RW Power Consumption) -> Bus Creator1/1  "RW#1 Power Consumption"
  1-axis Reaction Wheel (RW#2)/2(RW Power Consumption) -> Bus Creator1/2  "RW#2 Power Consumption"
  1-axis Reaction Wheel (RW#3)/2(RW Power Consumption) -> Bus Creator1/3  "RW#3 Power Consumption"
  1-axis Reaction Wheel (RW#3)/3(Motor Angular Velocity (rad/s)) -> Bus Creator2/3  "RW#3 Motor Angular Velocity (rad/s)"
  1-axis Reaction Wheel (RW#1)/3(Motor Angular Velocity (rad/s)) -> Bus Creator2/1  "RW#1 Motor Angular Velocity (rad/s)"
  1-axis Reaction Wheel (RW#2)/3(Motor Angular Velocity (rad/s)) -> Bus Creator2/2  "RW#2 Motor Angular Velocity (rad/s)"
  Bus Creator1/1 -> RWs Power Status/1
  1-axis Reaction Wheel (RW#4)/1(RW Torque Out) -> Bus Creator/4  "RW#4 Torque Out (N.m)"
  1-axis Reaction Wheel (RW#4)/2(RW Power Consumption) -> Bus Creator1/4  "RW#4 Power Consumption"
  Bus Selector1/4 -> 1-axis Reaction Wheel (RW#4)/2(RW Bus Voltage (V))  "<Power Bus: RW#4 (signal 8)>"
  Demux/4 -> 1-axis Reaction Wheel (RW#4)/1(Command Torque [Body](N.m))
  Actuator Physical Matrix (3*4)/1 -> Matrix Multiply/1
  Matrix Multiply/1 -> RWs Torque Out (Nm)/1
  Bus Creator/1 -> Matrix Multiply/2
  1-axis Reaction Wheel (RW#4)/3(Motor Angular Velocity (rad/s)) -> Bus Creator2/4  "RW#4 Motor Angular Velocity (rad/s)"
  Bus Creator2/1 -> RWs Angular Velocity (rad/s)/1
  Actuator Allocation Matrix (4*3)/1 -> Matrix Multiply1/1
  Matrix Multiply1/1 -> [TorqueCommand]  "Torque Command (4*1)"
  [TorqueCommand] -> Demux/1  "Torque Command (4*1)"

== system ADCSSimulator/ADCS/ADCS Hardware/Actuators/Tri-axial Magnetorquer Model (MTQs)/Power Consumption Calculator ==
  note: $I_=\frac{V_{Bus}}{R} \\ P_{Consumption} =I V_{Bus}$
  Bus Voltage (V) : Inport
  |m/m_max| : Inport  Port=2
  1/R : Gain  Gain=1/satellite.MTQ.Resistance(3)
  Bus Creator : BusCreator  Inputs=2
  Product : Product
  Product1 : Product
  Power Consumption : Outport
  wires:
  |m/m_max|/1 -> Product1/1
  Product1/1 -> Product/1, Bus Creator/1  "Current (A)"
  Bus Creator/1 -> Power Consumption/1
  Bus Voltage (V)/1 -> Product/2, 1/R/1
  Product/1 -> Bus Creator/2  "Power Consumption (W)"
  1/R/1 -> Product1/2

== system ADCSSimulator/ADCS/ADCS Hardware/Actuators/Tri-axial Magnetorquer Model (MTQs)/Power Consumption Calculator1 ==
  note: $I_=\frac{V_{Bus}}{R} \\ P_{Consumption} =I V_{Bus}$
  Bus Voltage (V) : Inport
  |m/m_max| : Inport  Port=2
  1/R : Gain  Gain=1/satellite.MTQ.Resistance(2)
  Bus Creator : BusCreator  Inputs=2
  Product : Product
  Product1 : Product
  Power Consumption : Outport
  wires:
  |m/m_max|/1 -> Product1/1
  Product1/1 -> Product/1, Bus Creator/1  "Current (A)"
  Bus Creator/1 -> Power Consumption/1
  Bus Voltage (V)/1 -> Product/2, 1/R/1
  Product/1 -> Bus Creator/2  "Power Consumption (W)"
  1/R/1 -> Product1/2

== system ADCSSimulator/ADCS/ADCS Hardware/Actuators/Tri-axial Magnetorquer Model (MTQs)/Power Consumption Calculator2 ==
  note: $I_=\frac{V_{Bus}}{R} \\ P_{Consumption} =I V_{Bus}$
  Bus Voltage (V) : Inport
  |m/m_max| : Inport  Port=2
  1/R : Gain  Gain=1/satellite.MTQ.Resistance(1)
  Bus Creator : BusCreator  Inputs=2
  Product : Product
  Product1 : Product
  Power Consumption : Outport
  wires:
  Bus Voltage (V)/1 -> Product/2, 1/R/1
  Product1/1 -> Product/1, Bus Creator/1  "Current (A)"
  Bus Creator/1 -> Power Consumption/1
  Product/1 -> Bus Creator/2  "Power Consumption (W)"
  |m/m_max|/1 -> Product1/1
  1/R/1 -> Product1/2

== system ADCSSimulator/ADCS/ADCS Hardware/Sensors/Analog Magnetometer Model/Init Data Wrapper ==
  Real Data : Inport
  Initial Value : Inport  Port=2
  Clock : Clock
  Switch : Switch  Threshold=1  SaturateOnIntegerOverflow=off  InputSameDT=off
  Wrapped Data : Outport
  wires:
  Switch/1 -> Wrapped Data/1
  Initial Value/1 -> Switch/3
  Real Data/1 -> Switch/1
  Clock/1 -> Switch/2

== system ADCSSimulator/ADCS/ADCS Hardware/Sensors/Analog Magnetometer Model/Power Consumption Calculator ==
  note: $I_=\frac{V_{Bus}}{R} \\ P_{Consumption} =I V_{Bus}$
  Bus Voltage (V) : Inport
  Bus Creator : BusCreator  Inputs=2
  Gain2 : Gain  Gain=1/(satellite.MM.NominalVoltage^2/satellite.MM.NominalPower)
  Product : Product
  MM Power Consumption : Outport
  wires:
  Product/1 -> Bus Creator/2  "Power Consumption (W)"
  Bus Creator/1 -> MM Power Consumption/1
  Gain2/1 -> Bus Creator/1, Product/1  "Current (A)"
  Bus Voltage (V)/1 -> Product/2, Gain2/1

== system ADCSSimulator/ADCS/ADCS Hardware/Sensors/Digital Magnetometer Model/Init Data Wrapper ==
  Real Data : Inport
  Initial Value : Inport  Port=2
  Clock : Clock
  Switch : Switch  Threshold=1  SaturateOnIntegerOverflow=off  InputSameDT=off
  Wrapped Data : Outport
  wires:
  Clock/1 -> Switch/2
  Real Data/1 -> Switch/1
  Initial Value/1 -> Switch/3
  Switch/1 -> Wrapped Data/1

== system ADCSSimulator/ADCS/ADCS Hardware/Sensors/Digital Magnetometer Model/Power Consumption Calculator ==
  note: $I_=\frac{V_{Bus}}{R} \\ P_{Consumption} =I V_{Bus}$
  Bus Voltage (V) : Inport
  Bus Creator : BusCreator  Inputs=2
  Gain2 : Gain  Gain=1/(satellite.MM.NominalVoltage^2/satellite.MM.NominalPower)
  Product : Product
  MM Power Consumption : Outport
  wires:
  Bus Voltage (V)/1 -> Gain2/1, Product/2
  Gain2/1 -> Product/1, Bus Creator/1  "Current (A)"
  Bus Creator/1 -> MM Power Consumption/1
  Product/1 -> Bus Creator/2  "Power Consumption (W)"

== system ADCSSimulator/ADCS/ADCS Hardware/Sensors/GNSS Receiver Model/Gauss-Markov ==
  Correlation Time Gain : Gain  Gain=1/satellite.GPS.Velocity.CorrelationTime
  Integrator : Integrator
  Noise Scaling Gain : Gain  Gain=sqrt(2 *satellite.GPS.Velocity.NoiseSTDDEV^2 / satellite.GPS.Velocity.CorrelationTime)
  Random Number : RandomNumber  Variance=satellite.GPS.Frequency  SampleTime=1/satellite.GPS.Frequency
  Sum : Sum  Inputs=|+-
  Correlated Noise Out : Outport
  wires:
  Random Number/1 -> Noise Scaling Gain/1
  Noise Scaling Gain/1 -> Sum/1
  Sum/1 -> Integrator/1
  Integrator/1 -> Correlated Noise Out/1, Correlation Time Gain/1
  Correlation Time Gain/1 -> Sum/2

== system ADCSSimulator/ADCS/ADCS Hardware/Sensors/GNSS Receiver Model/Gauss-Markov1 ==
  Correlation Time Gain : Gain  Gain=1/satellite.GPS.Velocity.CorrelationTime
  Integrator : Integrator
  Noise Scaling Gain : Gain  Gain=sqrt(2 *satellite.GPS.Velocity.NoiseSTDDEV^2 / satellite.GPS.Velocity.CorrelationTime)
  Random Number : RandomNumber  Variance=satellite.GPS.Frequency  SampleTime=1/satellite.GPS.Frequency
  Random Number1 : RandomNumber  Variance=satellite.GPS.Frequency  SampleTime=1/satellite.GPS.Frequency
  Sum : Sum  Inputs=|+-
  Correlated Noise Out : Outport
  wires:
  Correlation Time Gain/1 -> Sum/2
  Integrator/1 -> Correlation Time Gain/1, Correlated Noise Out/1
  Sum/1 -> Integrator/1
  Noise Scaling Gain/1 -> Sum/1
  Random Number1/1 -> Noise Scaling Gain/1

== system ADCSSimulator/ADCS/ADCS Hardware/Sensors/GNSS Receiver Model/Gauss-Markov2 ==
  Correlation Time Gain : Gain  Gain=1/satellite.GPS.Velocity.CorrelationTime
  Integrator : Integrator
  Noise Scaling Gain : Gain  Gain=sqrt(2 *satellite.GPS.Velocity.NoiseSTDDEV^2 / satellite.GPS.Velocity.CorrelationTime)
  Random Number : RandomNumber  Variance=satellite.GPS.Frequency  SampleTime=1/satellite.GPS.Frequency
  Random Number1 : RandomNumber  Variance=satellite.GPS.Frequency  SampleTime=1/satellite.GPS.Frequency
  Sum : Sum  Inputs=|+-
  Correlated Noise Out : Outport
  wires:
  Random Number1/1 -> Noise Scaling Gain/1
  Noise Scaling Gain/1 -> Sum/1
  Sum/1 -> Integrator/1
  Integrator/1 -> Correlated Noise Out/1, Correlation Time Gain/1
  Correlation Time Gain/1 -> Sum/2

== system ADCSSimulator/ADCS/ADCS Hardware/Sensors/GNSS Receiver Model/Gauss-Markov3 ==
  Correlation Time Gain : Gain  Gain=1/satellite.GPS.Position.CorrelationTime
  Integrator : Integrator
  Noise Scaling Gain : Gain  Gain=sqrt(2 *satellite.GPS.Position.NoiseSTDDEV^2 / satellite.GPS.Position.CorrelationTime)
  Random Number : RandomNumber  Variance=satellite.GPS.Frequency  SampleTime=1/satellite.GPS.Frequency
  Sum : Sum  Inputs=|+-
  Correlated Noise Out : Outport
  wires:
  Correlation Time Gain/1 -> Sum/2
  Integrator/1 -> Correlation Time Gain/1, Correlated Noise Out/1
  Sum/1 -> Integrator/1
  Noise Scaling Gain/1 -> Sum/1
  Random Number/1 -> Noise Scaling Gain/1

== system ADCSSimulator/ADCS/ADCS Hardware/Sensors/GNSS Receiver Model/Gauss-Markov4 ==
  Correlation Time Gain : Gain  Gain=1/satellite.GPS.Position.CorrelationTime
  Integrator : Integrator
  Noise Scaling Gain : Gain  Gain=sqrt(2 *satellite.GPS.Position.NoiseSTDDEV^2 / satellite.GPS.Position.CorrelationTime)
  Random Number : RandomNumber  Variance=satellite.GPS.Frequency  SampleTime=1/satellite.GPS.Frequency
  Random Number1 : RandomNumber  Variance=satellite.GPS.Frequency  SampleTime=1/satellite.GPS.Frequency
  Sum : Sum  Inputs=|+-
  Correlated Noise Out : Outport
  wires:
  Random Number1/1 -> Noise Scaling Gain/1
  Noise Scaling Gain/1 -> Sum/1
  Sum/1 -> Integrator/1
  Integrator/1 -> Correlated Noise Out/1, Correlation Time Gain/1
  Correlation Time Gain/1 -> Sum/2

== system ADCSSimulator/ADCS/ADCS Hardware/Sensors/GNSS Receiver Model/Gauss-Markov5 ==
  Correlation Time Gain : Gain  Gain=1/satellite.GPS.Position.CorrelationTime
  Integrator : Integrator
  Noise Scaling Gain : Gain  Gain=sqrt(2 *satellite.GPS.Position.NoiseSTDDEV^2 / satellite.GPS.Position.CorrelationTime)
  Random Number : RandomNumber  Variance=satellite.GPS.Frequency  SampleTime=1/satellite.GPS.Frequency
  Random Number1 : RandomNumber  Variance=satellite.GPS.Frequency  SampleTime=1/satellite.GPS.Frequency
  Sum : Sum  Inputs=|+-
  Correlated Noise Out : Outport
  wires:
  Correlation Time Gain/1 -> Sum/2
  Integrator/1 -> Correlation Time Gain/1, Correlated Noise Out/1
  Sum/1 -> Integrator/1
  Noise Scaling Gain/1 -> Sum/1
  Random Number1/1 -> Noise Scaling Gain/1

== system ADCSSimulator/ADCS/ADCS Hardware/Sensors/GNSS Receiver Model/Power Consumption Calculator ==
  note: $I_=\frac{V_{Bus}}{R} \\ P_{Consumption} =I V_{Bus}$
  Bus Voltage (V) : Inport
  Bus Creator : BusCreator  Inputs=2
  Gain2 : Gain  Gain=1/(satellite.GPS.NominalVoltage^2/satellite.GPS.NominalPower)
  Product : Product
  GPS Power Consumption : Outport
  wires:
  Bus Voltage (V)/1 -> Gain2/1, Product/2
  Gain2/1 -> Product/1, Bus Creator/1  "Current (A)"
  Bus Creator/1 -> GPS Power Consumption/1
  Product/1 -> Bus Creator/2  "Power Consumption (W)"

== system ADCSSimulator/ADCS/ADCS Hardware/Sensors/Gyroscope Model/Init Data Wrapper ==
  Real Data : Inport
  Initial Value : Inport  Port=2
  Clock : Clock
  Switch : Switch  Threshold=1  SaturateOnIntegerOverflow=off  InputSameDT=off
  Wrapped Data : Outport
  wires:
  Clock/1 -> Switch/2
  Real Data/1 -> Switch/1
  Initial Value/1 -> Switch/3
  Switch/1 -> Wrapped Data/1
